simulink subsystem "Gyro_Angles_sub"  (R2023b)
settings: Solver=VariableStepAuto  StartTime=0.0  StopTime=10.0  RelTol=1e-3
undefined symbols (not defined in the file): Auto_Starting_Position, Gyro_Calibration_Auto_Center, Gyro_Calibration_Auto_Left, Gyro_Calibration_Auto_Right, Gyro_Calibration_Default, Gyro_Calibration_Reset_Flag
libraries: simulink_extras x1, simulink x1
settings Model: Creator=ander  LastModifiedBy=ander

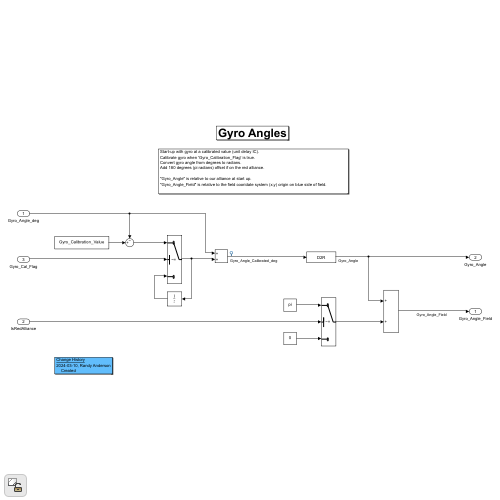
[thumbnail: Simulink's stored preview of the top-level diagram]
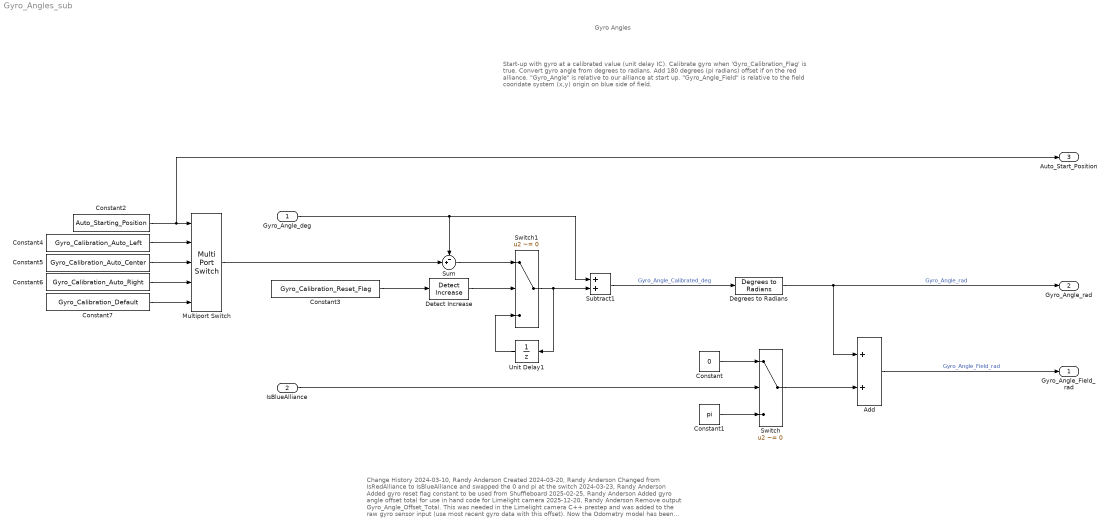
== system Gyro_Angles_sub ==
  note: Gyro Angles
  note: Start-up with gyro at a calibrated value (unit delay IC).
      | Calibrate gyro when 'Gyro_Calibration_Flag' is true.
      | Convert gyro angle from degrees to radians.
      | Add 180 degrees (pi radians) offset if on the red alliance.
      |
      | "Gyro_Angle" is relative to our alliance at start up.
      | "Gyro_Angle_Field" is relative to the field cooridate system (x,y) origin on blue side of field.
  note: Change History
      | 2024-03-10, Randy Anderson
      | Created
      | 2024-03-20, Randy Anderson
      | Changed from IsRedAlliance to IsBlueAlliance and swapped the 0 and pi at the switch
      | 2024-03-23, Randy Anderson
      | Added gyro reset flag constant to be used from Shuffleboard
      | 2025-02-25, Randy Anderson
      | Added gyro angle offset total for use in hand code for Limelight camera
      | 2025-12-20, Randy Anderson
      | Remove output Gyro_Angle_Offset_Total. This was needed in the Limelight camera C++ prestep and was added to the raw gyro
      | sensor input (use most recent gyro data with this offset). Now the Odometry model has been split out and runs before the Limelight
      | camera prestep, so we can instead use Gyro_Angle_Field_rad (with conversion to degrees in C++) which already includes the offsets.
  Gyro_Angle_deg : Inport
  IsBlueAlliance : Inport  Port=2
  Add : Sum
  Constant : Constant  Value=0
  Constant1 : Constant  Value=pi
  Constant2 : Constant  Value=Auto_Starting_Position  OutDataTypeStr=double
  Constant3 : Constant  Value=Gyro_Calibration_Reset_Flag
  Constant4 : Constant  Value=Gyro_Calibration_Auto_Left  OutDataTypeStr=double
  Constant5 : Constant  Value=Gyro_Calibration_Auto_Center  OutDataTypeStr=double
  Constant6 : Constant  Value=Gyro_Calibration_Auto_Right  OutDataTypeStr=double
  Constant7 : Constant  Value=Gyro_Calibration_Default  OutDataTypeStr=double
  Degrees to Radians : simulink_extras/Transformations/Degrees to Radians
  Detect Increase : simulink/Logic and Bit Operations/Detect Increase  vinit=0.0  OutDataTypeStr=boolean
  Multiport Switch : MultiPortSwitch  DataPortForDefault=Additional data port  SaturateOnIntegerOverflow=off  InputSameDT=off
  Subtract1 : Sum
  Sum : Sum  Inputs=-+|
  Switch : Switch  Criteria=u2 ~= 0  SaturateOnIntegerOverflow=off  InputSameDT=off
  Switch1 : Switch  Criteria=u2 ~= 0  SaturateOnIntegerOverflow=off  InputSameDT=off
  Unit Delay1 : UnitDelay  InitialCondition=Gyro_Calibration_Default  SampleTime=-1  HasFrameUpgradeWarning=on
  Gyro_Angle_Field_rad : Outport
  Gyro_Angle_rad : Outport  Port=2
  Auto_Start_Position : Outport  Port=3
  wires:
  Add/1 -> Gyro_Angle_Field_rad/1  "Gyro_Angle_Field_rad"
  Degrees to Radians/1 -> Gyro_Angle_rad/1, Add/1  "Gyro_Angle_rad"
  IsBlueAlliance/1 -> Switch/2
  Constant/1 -> Switch/1
  Constant1/1 -> Switch/3
  Unit Delay1/1 -> Switch1/3
  Switch1/1 -> Subtract1/2, Unit Delay1/1
  Sum/1 -> Switch1/1
  Subtract1/1 -> Degrees to Radians/1  "Gyro_Angle_Calibrated_deg"
  Gyro_Angle_deg/1 -> Sum/1, Subtract1/1
  Multiport Switch/1 -> Sum/2
  Switch/1 -> Add/2
  Constant3/1 -> Detect Increase/1
  Detect Increase/1 -> Switch1/2
  Constant2/1 -> Multiport Switch/1, Auto_Start_Position/1
  Constant5/1 -> Multiport Switch/3
  Constant6/1 -> Multiport Switch/4
  Constant4/1 -> Multiport Switch/2
  Constant7/1 -> Multiport Switch/5
